simulink model "ferrari_sym"  (R2023a)
settings: Solver=VariableStepAuto  StartTime=0.0  StopTime=20  RelTol=1e-7
values from neighbouring files (symbols this model uses):
  Ce = C*C1*delayNet    [ferrari_matlab.m]
  desat = 1/(s+0.01)    [ferrari_matlab.m]
  Fr = 1/(1*s+1)    [ferrari_matlab.m]
  Fr1 = 1/(2*s+1)    [ferrari_matlab.m]
  gain = 110    [ferrari_matlab.m]
  H = (s^2+(omega_n)^2)/(s^2 + 2*zita*omega_n*s + omega_n^2)    [ferrari_matlab.m]
  Pe = W1e + ds*W2e    [ferrari_matlab.m]
settings Model: Creator=aless  LastModifiedBy=aless
settings SolverCC: ZeroCrossAlgorithm=Adaptive
settings DebuggingCC: IgnoredZcDiagnostic=none

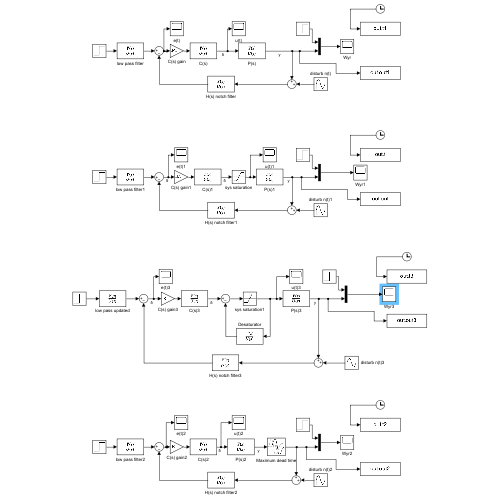
[thumbnail: Simulink's stored preview of the top-level diagram]
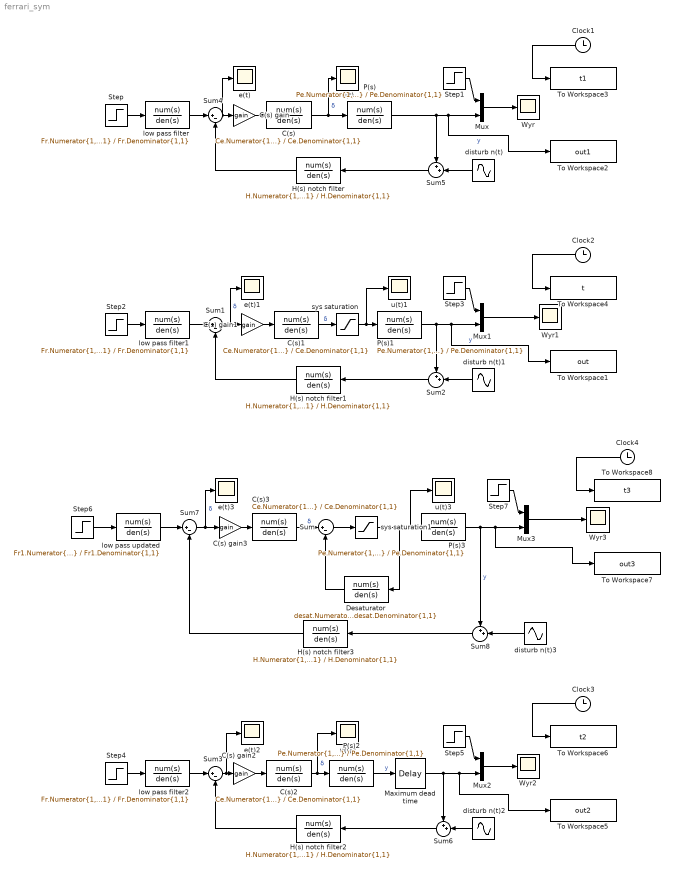
== system ferrari_sym ==
  C(s){,1..3} (4 alike) : TransferFcn  Numerator=Ce.Numerator{1,1}  Denominator=Ce.Denominator{1,1}
  C(s) gain{,1..3} (4 alike) : Gain  Gain=gain
  Clock{1..4} (4 alike) : Clock
  Desaturator : TransferFcn  Numerator=desat.Numerator{1,1}  Denominator=desat.Denominator{1,1}
  H(s) notch filter{,1..3} (4 alike) : TransferFcn  Numerator=H.Numerator{1,1}  Denominator=H.Denominator{1,1}
  Maximum dead time : TransportDelay  DelayTime=0.3  PadeOrder=3
  Mux{,1..3} (4 alike) : Mux  Inputs=2
  P(s){,1..3} (4 alike) : TransferFcn  Numerator=Pe.Numerator{1,1}  Denominator=Pe.Denominator{1,1}
  Step{,2,4,6} (4 alike) : Step  Time=0  SampleTime=0
  Step{1,3,5,7} (4 alike) : Step  SampleTime=0
  Sum{,1,3..4,7} (5 alike) : Sum  Inputs=|+-
  Sum{2,5..6,8} (4 alike) : Sum  Inputs=++|
  To Workspace1 : ToWorkspace  VariableName=out  SaveFormat=Timeseries
  To Workspace2 : ToWorkspace  VariableName=out1  SaveFormat=Timeseries
  To Workspace3 : ToWorkspace  VariableName=t1  SaveFormat=Timeseries
  To Workspace4 : ToWorkspace  VariableName=t  SaveFormat=Timeseries
  To Workspace5 : ToWorkspace  VariableName=out2  SaveFormat=Timeseries
  To Workspace6 : ToWorkspace  VariableName=t2  SaveFormat=Timeseries
  To Workspace7 : ToWorkspace  VariableName=out3  SaveFormat=Timeseries
  To Workspace8 : ToWorkspace  VariableName=t3  SaveFormat=Timeseries
  Wyr{,1..3} (4 alike) : Scope
  disturb n(t){,1..3} (4 alike) : Sin  Amplitude=4*pi/180  Frequency=2*3*pi  SampleTime=0
  e(t){,1..3} (4 alike) : Scope
  low pass filter : TransferFcn  Numerator=Fr.Numerator{1,1}  Denominator=Fr.Denominator{1,1}
  low pass filter1 : TransferFcn  Numerator=Fr.Numerator{1,1}  Denominator=Fr.Denominator{1,1}
  low pass filter2 : TransferFcn  Numerator=Fr.Numerator{1,1}  Denominator=Fr.Denominator{1,1}
  low pass updated : TransferFcn  Numerator=Fr1.Numerator{1,1}  Denominator=Fr1.Denominator{1,1}
  sys saturation : Saturate  UpperLimit=0.0025  LowerLimit=-0.0025
  sys saturation1 : Saturate  UpperLimit=0.0025  LowerLimit=-0.0025
  u(t){,1..3} (4 alike) : Scope
  wires:
  Clock1/1 -> To Workspace3/1
  Mux/1 -> Wyr/1
  disturb n(t)/1 -> Sum5/2
  low pass filter/1 -> Sum4/1
  Step1/1 -> Mux/1
  Step/1 -> low pass filter/1
  C(s) gain/1 -> C(s)/1
  Sum5/1 -> H(s) notch filter/1
  H(s) notch filter/1 -> Sum4/2
  H(s) notch filter1/1 -> Sum1/2
  Sum2/1 -> H(s) notch filter1/1
  Clock2/1 -> To Workspace4/1
  low pass filter1/1 -> Sum1/1
  P(s)1/1 -> Mux1/2, To Workspace1/1, Sum2/1  "y"
  Step2/1 -> low pass filter1/1
  Mux1/1 -> Wyr1/1
  disturb n(t)1/1 -> Sum2/2
  H(s) notch filter2/1 -> Sum3/2
  Sum6/1 -> H(s) notch filter2/1
  C(s) gain2/1 -> C(s)2/1
  Clock3/1 -> To Workspace6/1
  low pass filter2/1 -> Sum3/1
  Step5/1 -> Mux2/1
  Step4/1 -> low pass filter2/1
  C(s)2/1 -> u(t)2/1, P(s)2/1  "δ"
  Mux2/1 -> Wyr2/1
  disturb n(t)2/1 -> Sum6/2
  P(s)2/1 -> Maximum dead time/1  "y"
  Maximum dead time/1 -> To Workspace5/1, Mux2/2, Sum6/1
  C(s)/1 -> u(t)/1, P(s)/1  "δ"
  P(s)/1 -> Sum5/1, To Workspace2/1, Mux/2  "y"
  C(s) gain1/1 -> C(s)1/1
  Step3/1 -> Mux1/1
  Sum1/1 -> C(s) gain1/1, e(t)1/1  "δ"
  Sum4/1 -> e(t)/1, C(s) gain/1
  Sum3/1 -> e(t)2/1, C(s) gain2/1
  Sum7/1 -> C(s) gain3/1, e(t)3/1  "δ"
  C(s) gain3/1 -> C(s)3/1
  disturb n(t)3/1 -> Sum8/2
  Clock4/1 -> To Workspace8/1
  Step7/1 -> Mux3/1
  P(s)3/1 -> Mux3/2, To Workspace7/1, Sum8/1  "y"
  Mux3/1 -> Wyr3/1
  H(s) notch filter3/1 -> Sum7/2
  low pass updated/1 -> Sum7/1
  Sum8/1 -> H(s) notch filter3/1
  Step6/1 -> low pass updated/1
  C(s)1/1 -> sys saturation/1  "δ"
  sys saturation/1 -> u(t)1/1, P(s)1/1
  sys saturation1/1 -> Desaturator/1, u(t)3/1, P(s)3/1
  Desaturator/1 -> Sum/2
  C(s)3/1 -> Sum/1  "δ"
  Sum/1 -> sys saturation1/1
